simulink model "operational_space_inverse_dynamics"  (R2024b)
settings: Solver=VariableStepAuto  StartTime=0.0  StopTime=24*5+6  RelTol=1e-3
undefined symbols (not defined in the file): Kd_op, Ki_op, Kp_op, ml, q0, Tc
libraries: slpidlib x1
settings Model: Creator=storm  LastModifiedBy=giaco
settings OptimizationCC: ReuseModelBlockBuffer=off
settings DebuggingCC: UnconnectedInputMsg=warning  UnconnectedOutputMsg=warning  UnconnectedLineMsg=warning
settings ModelReferenceCC: EnableRefExpFcnMdlSchedulingChecks=on
settings RTWCC: GPUComputeCapability=3.5  DLArmComputeVersion=19.05

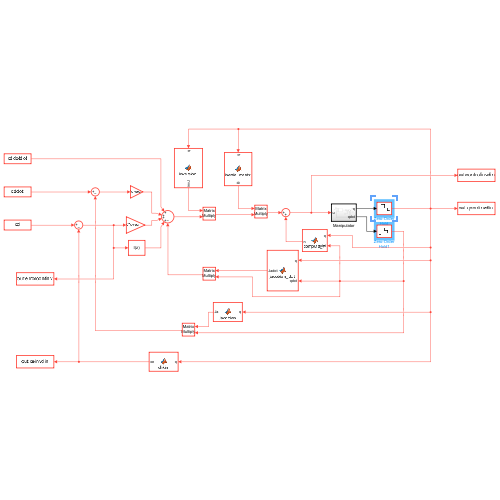
[thumbnail: Simulink's stored preview of the top-level diagram]
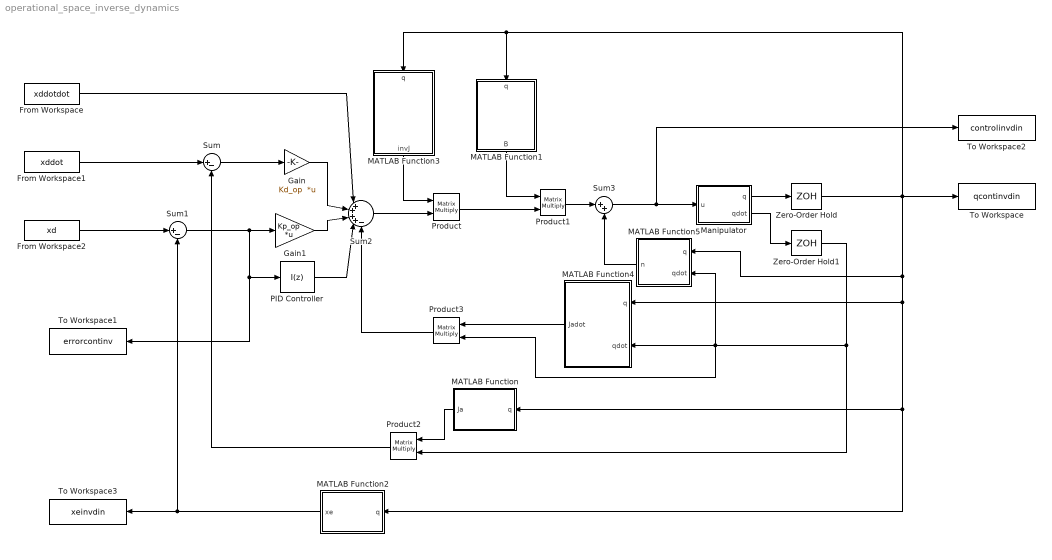
== system operational_space_inverse_dynamics ==
  From Workspace : FromWorkspace  VariableName=xddotdot  SampleTime=Tc
  From Workspace1 : FromWorkspace  VariableName=xddot  SampleTime=Tc
  From Workspace2 : FromWorkspace  VariableName=xd  SampleTime=Tc
  Gain : Gain  Gain=Kd_op  Multiplication=Matrix(K*u) (u vector)
  Gain1 : Gain  Gain=Kp_op  Multiplication=Matrix(K*u) (u vector)
  MATLAB Function : MATLAB Function  TreatAsAtomicUnit=on
  MATLAB Function1 : MATLAB Function  TreatAsAtomicUnit=on
  MATLAB Function2 : MATLAB Function  TreatAsAtomicUnit=on
  MATLAB Function3 : MATLAB Function  TreatAsAtomicUnit=on
  MATLAB Function4 : MATLAB Function  TreatAsAtomicUnit=on
  MATLAB Function5 : MATLAB Function  TreatAsAtomicUnit=on
  Manipulator : Subsystem
  PID Controller : slpidlib/PID Controller  Controller=I  Form=Parallel  TimeDomain=Discrete-time  UseExternalTs=off  SampleTime=-1  IntegratorMethod=Forward Euler  FilterMethod=Forward Euler  ControllerParametersSource=internal  P=1  I=diag(Ki_op)  UseKiTs=off  D=0  UseExternalDerivativeSource=off  N=100  UseFilter=on  TunerSelectOption=Transfer Function Based (PID Tuner App)  InitialConditionSource=internal  InitialConditionForIntegrator=0  InitialConditionForFilter=0  DifferentiatorICPrevScaledInput=0  ExternalReset=none  TrackingMode=off  Kt=1  LimitOutput=off  SatLimitsSource=internal  UpperSaturationLimit=inf  LowerSaturationLimit=-inf  LinearizeAsGain=on  AntiWindupMode=none  Kb=1  LimitIntegrator=off  UpperIntegratorSaturationLimit=inf  LowerIntegratorSaturationLimit=-inf  POutMin=[]  POutMax=[]  IOutMin=[]  IOutMax=[]  DOutMin=[]  DOutMax=[]  NOutMin=[]  NOutMax=[]  SumOutMin=[]  SumOutMax=[]  SaturationOutMin=[]  SaturationOutMax=[]  PParamMin=[]  PParamMax=[]  IParamMin=[]  IParamMax=[]  DParamMin=[]  DParamMax=[]  NParamMin=[]  NParamMax=[]  KbParamMin=[]  KbParamMax=[]  KtParamMin=[]  KtParamMax=[]  KbOutMin=[]  KbOutMax=[]  KtOutMin=[]  KtOutMax=[]  IntegratorOutMin=[]  IntegratorOutMax=[]  FilterOutMin=[]  FilterOutMax=[]  SumI1OutMin=[]  SumI1OutMax=[]  SumI2OutMin=[]  SumI2OutMax=[]  SumI3OutMin=[]  SumI3OutMax=[]  SumI4OutMin=[]  SumI4OutMax=[]  SumDOutMin=[]  SumDOutMax=[]  DifferentiatorOutMin=[]  DifferentiatorOutMax=[]  FilterDiffOutCoefMin=[]  FilterDiffOutCoefMax=[]  ReciprocalOutMin=[]  ReciprocalOutMax=[]  SumDenOutMin=[]  SumDenOutMax=[]  SumNumOutMin=[]  SumNumOutMax=[]  DivideOutMin=[]  DivideOutMax=[]  UdiffTsProdOutMin=[]  UdiffTsProdOutMax=[]  NTsProdOutMin=[]  NTsProdOutMax=[]  UintegralTsProdOutMin=[]  UintegralTsProdOutMax=[]  UngainTsProdOutMin=[]  UngainTsProdOutMax=[]  ClampingZeroOutDataTypeStr=Inherit: Inherit via back propagation  ClampingZeroOutMin=[]  ClampingZeroOutMax=[]  FilterDenConstantOutDataTypeStr=Inherit: Inherit via back propagation  FilterDenConstantOutMin=[]  FilterDenConstantOutMax=[]  PCopyOutDataTypeStr=Inherit: Inherit via back propagation  PCopyOutMin=[]  PCopyOutMax=[]  NCopyOutDataTypeStr=Inherit: Inherit via back propagation  NCopyOutMin=[]  NCopyOutMax=[]  IntegratorContinuousStateAttributes=''  IntegratorStateMustResolveToSignalObject=off  IntegratorRTWStateStorageClass=Auto  FilterContinuousStateAttributes=''  FilterStateMustResolveToSignalObject=off  FilterRTWStateStorageClass=Auto  ParallelPVariant=Disabled  IdealPVariant=Disabled  IVariant=InternalParameters  DVariant=Disabled  IntegratorVariant=Discrete  SatVariant=Disabled  AWVariant=Passthrough  PCopyVariant=Disabled  TRVariant=Disabled  FdbkBlocksVariant=Forward  IdealPFdbkVariant=Disabled  SatFdbkVariant=Disabled  DerivativeFilterVariant=Disabled  NVariant=Disabled  NCopyVariant=Disabled_SignalSpec  FilterICVariant=Disabled  IntegratorICVariant=InternalICs  ExternalResetVariant=Disabled  TRSumVariant=Passthrough  SumFdbkVariant=Disabled  SumVariant=Passthrough_I  TsampFilterVariant=InternalTs  TsampNgainVariant=Passthrough  TsampIntegralVariant=Disabled_SignalSpec  ExternalSaturationOutDataTypeStr=Inherit: Same as second input  DerivativeSourceVariant=Disabled  PreIntVariant=InternalPreInt
  Product{,1..3} (4 alike) : Product  Multiplication=Matrix(*)
  Sum : Sum  Inputs=|+-
  Sum1 : Sum  Inputs=|+-
  Sum2 : Sum  Inputs=|++++-
  Sum3 : Sum  Inputs=|++
  To Workspace : ToWorkspace  VariableName=qcontinvdin  SaveFormat=Structure With Time  SampleTime=-1
  To Workspace1 : ToWorkspace  VariableName=errorcontinv  SaveFormat=Structure With Time  SampleTime=-1
  To Workspace2 : ToWorkspace  VariableName=controlinvdin  SaveFormat=Structure With Time  SampleTime=-1
  To Workspace3 : ToWorkspace  VariableName=xeinvdin  SaveFormat=Structure With Time  SampleTime=-1
  Zero-Order Hold : ZeroOrderHold  SampleTime=Tc
  Zero-Order Hold1 : ZeroOrderHold  SampleTime=Tc
  wires:
  From Workspace1/1 -> Sum/1
  From Workspace2/1 -> Sum1/1
  Sum1/1 -> PID Controller/1, To Workspace1/1, Gain1/1
  Sum/1 -> Gain/1
  From Workspace/1 -> Sum2/1
  MATLAB Function3/1(invJ) -> Product/1
  Sum2/1 -> Product/2
  MATLAB Function1/1(B) -> Product1/1
  Product/1 -> Product1/2
  Product1/1 -> Sum3/1
  Manipulator/1(q) -> Zero-Order Hold/1
  Zero-Order Hold/1 -> MATLAB Function3/1(q), MATLAB Function1/1(q), MATLAB Function5/1(q), MATLAB Function4/1(q), MATLAB Function/1(q), MATLAB Function2/1(q), To Workspace/1
  MATLAB Function/1(Ja) -> Product2/1
  Product2/1 -> Sum/2
  MATLAB Function2/1(xe) -> Sum1/2, To Workspace3/1
  MATLAB Function4/1(Jadot) -> Product3/1
  Product3/1 -> Sum2/5
  MATLAB Function5/1(n) -> Sum3/2
  Gain/1 -> Sum2/2
  Gain1/1 -> Sum2/3
  Sum3/1 -> To Workspace2/1, Manipulator/1(u)
  Manipulator/2(qdot) -> Zero-Order Hold1/1
  Zero-Order Hold1/1 -> Product3/2, MATLAB Function5/2(qdot), MATLAB Function4/2(qdot), Product2/2
  PID Controller/1 -> Sum2/4

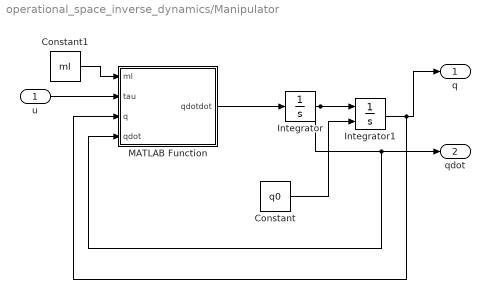
== system operational_space_inverse_dynamics/Manipulator ==
  u : Inport
  Constant : Constant  Value=q0
  Constant1 : Constant  Value=ml
  Integrator : Integrator  InitialCondition=[0 0 0 0]'
  Integrator1 : Integrator  InitialConditionSource=external
  MATLAB Function : MATLAB Function  TreatAsAtomicUnit=on
  q : Outport
  qdot : Outport  Port=2
  wires:
  u/1 -> MATLAB Function/2(tau)
  Integrator/1 -> MATLAB Function/4(qdot), qdot/1, Integrator1/1
  Constant/1 -> Integrator1/2
  Integrator1/1 -> MATLAB Function/3(q), q/1
  Constant1/1 -> MATLAB Function/1(ml)
  MATLAB Function/1(qdotdot) -> Integrator/1

== matlab function operational_space_inverse_dynamics/MATLAB Function2 ==
  data: q input; xe output
function xe = dirkin(q)
% Pose in base coordinates, ordered as [x; y; z; phi].
a1=0.5;
a2=a1;
d0=1;

xe=[a1*cos(q(1))+a2*cos(q(1)+q(2));...
    a1*sin(q(1))+a2*sin(q(1)+q(2));...
    d0+q(3);...
    q(1)+q(2)+q(4)];
end

== matlab function operational_space_inverse_dynamics/MATLAB Function ==
  data: q input; Ja output
function Ja = Jacobian(q)
% Map joint rates to [x_dot; y_dot; z_dot; phi_dot].
a1=0.5;
a2=a1;
d0=1;

Ja= [-a1*sin(q(1))-a2*sin(q(1)+q(2)),-a2*sin(q(1)+q(2)),0,0;...
    a1*cos(q(1))+a2*cos(q(1)+q(2)),a2*cos(q(1)+q(2)),0,0;...
    0,0,1,0;...
    1,1,0,1];
end

== matlab function operational_space_inverse_dynamics/MATLAB Function4 ==
  data: q input; Jadot output; qdot input
function Jadot = jacobian_dot(q,qdot)
% Only the planar rows change with the joint angles.

a1=0.5;
a2=a1;

Jadot= [qdot(1)*(-a1*cos(q(1)))-(qdot(1)+qdot(2))*a2*cos(q(1)+q(2)),(qdot(1)+qdot(2))*(-a2*cos(q(1)+q(2))),0,0;...
    qdot(1)*(-a1*sin(q(1)))-(qdot(1)+qdot(2))*a2*sin(q(1)+q(2)),(qdot(1)+qdot(2))*(-a2*sin(q(1)+q(2))),0,0;...
    0,0,0,0;...
    0,0,0,0];

end

== matlab function operational_space_inverse_dynamics/MATLAB Function3 ==
  data: invJ output; q input
function invJ=inversion(q)
% Map the full pose correction back to joint space.

a1=0.5;
a2=a1;

J = [-a1*sin(q(1))-a2*sin(q(1)+q(2)),-a2*sin(q(1)+q(2)),0,0;...
      a1*cos(q(1))+a2*cos(q(1)+q(2)),a2*cos(q(1)+q(2)),0,0;...
      0,0,1,0;...
      1,1,0,1];

invJ=J^-1;

end

== matlab function operational_space_inverse_dynamics/MATLAB Function1 ==
  data: q input; B output
function B = inertia_matrix(q)
% Joint-space inertia for the controller model.

a1=0.5;
a2=0.5;
l1=0.25;
l2=0.25;
ml1=20;
ml2=20;
ml3=10;
Il1=4;
Il2=4;
Il4=1;
kr1=1;
kr2=1;
kr3=50;
kr4=20;
Im1=0.01;
Im2=0.01;
Im3=0.005;
Im4=0.001;

mhe=0; % Payload mass parameter [kg]

% Link and rotor Jacobians used to assemble the inertia matrix.
Jpl1=[-l1*sin(q(1)) 0 0 0;
    l1*cos(q(1)) 0 0 0;
    0 0 0 0];

Jpl2=[-a1*sin(q(1))-l2*sin(q(1)+q(2)),-l2*sin(q(1)+q(2)),0,0;
    a1*cos(q(1))+l2*cos(q(1)+q(2)),l2*cos(q(1)+q(2)),0,0;
    0,0,0,0];

Jpl4=[-a1*sin(q(1))-a2*sin(q(1)+q(2)),-a2*sin(q(1)+q(2)),0,0;
    a1*cos(q(1))+a2*cos(q(1)+q(2)),a2*cos(q(1)+q(2)),0,0;
    0,0,1,0];

Jol1=[zeros(2,4);
    1 0 0 0];

Jol2=[zeros(2,4);
    1 1 0 0];

Jol4=[zeros(2,4);
    1 1 0 1];

Jom1=[zeros(2,4);
    kr1 0 0 0];

Jom2=[zeros(2,4);
    1 kr2 0 0];

Jom3=[zeros(2,4);
    1 1 kr3 0];

Jom4=[zeros(2,4);
    1 1 0 kr4];

B=ml1*(Jpl1'*Jpl1)+Jol1'*Il1*Jol1+Jom1'*Im1*Jom1...
    +ml2*(Jpl2'*Jpl2)+Jol2'*Il2*Jol2+Jom2'*Im2*Jom2...
    +Jom3'*Im3*Jom3...
    +(mhe+ml3)*(Jpl4'*Jpl4)+Jol4'*Il4*Jol4+Jom4'*Im4*Jom4;

end

== matlab function operational_space_inverse_dynamics/MATLAB Function5 ==
  data: q input; n output; qdot input
function n = compute_n(q,qdot)
% Add the velocity and gravity terms used in inverse dynamics.

a1=0.5;
a2=0.5;
l1=0.25;
l2=0.25;
ml1=20;
ml2=20;
ml3=10;
Il1=4;
Il2=4;
Il4=1;
kr1=1;
kr2=1;
kr3=50;
kr4=20;
Im1=0.01;
Im2=0.01;
Im3=0.005;
Im4=0.001;
Fm1=0.00005;
Fm2=0.00005;
Fm3=0.01;
Fm4=0.005;

mhe=0; % Payload mass parameter [kg]

% Link and rotor Jacobians used to assemble the inertia matrix.
Jpl1=[-l1*sin(q(1)) 0 0 0;
       l1*cos(q(1)) 0 0 0;
       0 0 0 0];

Jpl2=[-a1*sin(q(1))-l2*sin(q(1)+q(2)),-l2*sin(q(1)+q(2)),0,0;
       a1*cos(q(1))+l2*cos(q(1)+q(2)),l2*cos(q(1)+q(2)),0,0;
       0,0,0,0];

Jpl4=[-a1*sin(q(1))-a2*sin(q(1)+q(2)),-a2*sin(q(1)+q(2)),0,0;
       a1*cos(q(1))+a2*cos(q(1)+q(2)),a2*cos(q(1)+q(2)),0,0;
       0,0,1,0];

Jol1=[zeros(2,4);
      1 0 0 0];

Jol2=[zeros(2,4);
      1 1 0 0];

Jol4=[zeros(2,4);
      1 1 0 1];

Jom1=[zeros(2,4);
      kr1 0 0 0];

Jom2=[zeros(2,4);
      1 kr2 0 0];

Jom3=[zeros(2,4);
      1 1 kr3 0];

Jom4=[zeros(2,4);
      1 1 0 kr4];

B=ml1*(Jpl1'*Jpl1)+Jol1'*Il1*Jol1+Jom1'*Im1*Jom1...
    +ml2*(Jpl2'*Jpl2)+Jol2'*Il2*Jol2+Jom2'*Im2*Jom2...
    +Jom3'*Im3*Jom3...
    +ml3*(Jpl4'*Jpl4)+Jol4'*Il4*Jol4+Jom4'*Im4*Jom4;

% Build the Coriolis matrix from the inertia derivatives.
c=zeros(4,4,4);

Jpl1dq1=[-l1*cos(q(1)) 0 0 0;
         -l1*sin(q(1)) 0 0 0;
          0 0 0 0];

Jpl1dq2=zeros(3,4);

Jpl2dq1=[-a1*cos(q(1))-l2*cos(q(1)+q(2)),-l2*cos(q(1)+q(2)),0,0;
         -a1*sin(q(1))-l2*sin(q(1)+q(2)),-l2*sin(q(1)+q(2)),0,0;
          0,0,0,0];

Jpl2dq2=[-l2*cos(q(1)+q(2)),-l2*cos(q(1)+q(2)),0,0;
         -l2*sin(q(1)+q(2)),-l2*sin(q(1)+q(2)),0,0;
          0,0,0,0];

Jpl4dq1=[-a1*cos(q(1))-a2*cos(q(1)+q(2)),-a2*cos(q(1)+q(2)),0,0;
         -a1*sin(q(1))-a2*sin(q(1)+q(2)),-a2*sin(q(1)+q(2)),0,0;
          0,0,0,0];

Jpl4dq2=[-a2*cos(q(1)+q(2)),-a2*cos(q(1)+q(2)),0,0;
         -a2*sin(q(1)+q(2)),-a2*sin(q(1)+q(2)),0,0;
          0,0,0,0];

dBdq1=ml1*(Jpl1dq1'*Jpl1+Jpl1'*Jpl1dq1)+ml2*(Jpl2dq1'*Jpl2+Jpl2'*Jpl2dq1)+ml3*(Jpl4dq1'*Jpl4+Jpl4'*Jpl4dq1);
dBdq2=ml1*(Jpl1dq2'*Jpl1+Jpl1'*Jpl1dq2)+ml2*(Jpl2dq2'*Jpl2+Jpl2'*Jpl2dq2)+ml3*(Jpl4dq2'*Jpl4+Jpl4'*Jpl4dq2);

c(1,1,2)=-ml2*a1*l2*sin(q(2))-ml3*a1*a2*sin(q(2));
c(1,2,2)=c(1,1,2);
c(2,1,1)=-c(1,1,2);

C=zeros(4,4);
    for i=1:4
        for j=1:4
            for k=1:4
                C(i,j)=c(i,j,k)*qdot(k);
            end
        end
    end

g = [0 0 9.81*(mhe+ml3) 0]';

Fv = diag([kr1^2*Fm1,kr2^2*Fm2,kr3^2*Fm3,kr4^2*Fm4]);

n = C*qdot+Fv*qdot+g;

== matlab function operational_space_inverse_dynamics/Manipulator/MATLAB Function ==
  data: ml input; qdotdot output; tau input; q input; qdot input
function qdotdot= Dinamica_diretta(ml,tau,q,qdot)
% Plant dynamics: subtract Coriolis, friction, and gravity before solving for acceleration.
a1=0.5;
a2=0.5;
l1=0.25;
l2=0.25;
ml1=20;
ml2=20;
ml3=10;
Il1=4;
Il2=4;
Il4=1;
kr1=1;
kr2=1;
kr3=50;
kr4=20;
Im1=0.01;
Im2=0.01;
Im3=0.005;
Im4=0.001;

Fm1=0.00005;
Fm2=0.00005;
Fm3=0.01;
Fm4=0.005;

mhe=4; % Payload mass parameter [kg]
% Link and rotor Jacobians used to assemble the inertia matrix.
Jpl1=[-l1*sin(q(1)) 0 0 0;
    l1*cos(q(1)) 0 0 0;
    0 0 0 0];

Jpl2=[-a1*sin(q(1))-l2*sin(q(1)+q(2)),-l2*sin(q(1)+q(2)),0,0;
    a1*cos(q(1))+l2*cos(q(1)+q(2)),l2*cos(q(1)+q(2)),0,0;
    0,0,0,0];

Jpl4=[-a1*sin(q(1))-a2*sin(q(1)+q(2)),-a2*sin(q(1)+q(2)),0,0;
    a1*cos(q(1))+a2*cos(q(1)+q(2)),a2*cos(q(1)+q(2)),0,0;
    0,0,1,0];

Jol1=[zeros(2,4);
    1 0 0 0];

Jol2=[zeros(2,4);
    1 1 0 0];

Jol4=[zeros(2,4);
    1 1 0 1];

Jom1=[zeros(2,4);
    kr1 0 0 0];

Jom2=[zeros(2,4);
    1 kr2 0 0];

Jom3=[zeros(2,4);
    1 1 kr3 0];

Jom4=[zeros(2,4);
    1 1 0 kr4];

B=ml1*(Jpl1'*Jpl1)+Jol1'*Il1*Jol1+Jom1'*Im1*Jom1...
    +ml2*(Jpl2'*Jpl2)+Jol2'*Il2*Jol2+Jom2'*Im2*Jom2...
    +Jom3'*Im3*Jom3...
    +(ml+ml3)*(Jpl4'*Jpl4)+Jol4'*Il4*Jol4+Jom4'*Im4*Jom4;

c=zeros(4,4,4);

Jpl1dq1=[-l1*cos(q(1)) 0 0 0;
    -l1*sin(q(1)) 0 0 0;
    0 0 0 0];

Jpl1dq2=zeros(3,4);

Jpl2dq1=[-a1*cos(q(1))-l2*cos(q(1)+q(2)),-l2*cos(q(1)+q(2)),0,0;
    -a1*sin(q(1))-l2*sin(q(1)+q(2)),-l2*sin(q(1)+q(2)),0,0;
    0,0,0,0];

Jpl2dq2=[-l2*cos(q(1)+q(2)),-l2*cos(q(1)+q(2)),0,0;
    -l2*sin(q(1)+q(2)),-l2*sin(q(1)+q(2)),0,0;
    0,0,0,0];

Jpl4dq1=[-a1*cos(q(1))-a2*cos(q(1)+q(2)),-a2*cos(q(1)+q(2)),0,0;
    -a1*sin(q(1))-a2*sin(q(1)+q(2)),-a2*sin(q(1)+q(2)),0,0;
    0,0,0,0];

Jpl4dq2=[-a2*cos(q(1)+q(2)),-a2*cos(q(1)+q(2)),0,0;
    -a2*sin(q(1)+q(2)),-a2*sin(q(1)+q(2)),0,0;
    0,0,0,0];

dBdq1=ml1*(Jpl1dq1'*Jpl1+Jpl1'*Jpl1dq1)+ml2*(Jpl2dq1'*Jpl2+Jpl2'*Jpl2dq1)+ml3*(Jpl4dq1'*Jpl4+Jpl4'*Jpl4dq1);
dBdq2=ml1*(Jpl1dq2'*Jpl1+Jpl1'*Jpl1dq2)+ml2*(Jpl2dq2'*Jpl2+Jpl2'*Jpl2dq2)+ml3*(Jpl4dq2'*Jpl4+Jpl4'*Jpl4dq2);

c(1,1,2)=-ml2*a1*l2*sin(q(2))-ml3*a1*a2*sin(q(2));
c(1,2,2)=c(1,1,2);
c(2,1,1)=-c(1,1,2);

C=zeros(4,4);
    for i=1:4
        for j=1:4
            for k=1:4
                C(i,j)=c(i,j,k)*qdot(k);
            end
        end
    end

g=[0 0 9.81*(ml+ml3) 0]';

Fv=diag([kr1^2*Fm1,kr2^2*Fm2,kr3^2*Fm3,kr4^2*Fm4]);
qdotdot=inv(B)*(tau-C*qdot-Fv*qdot-g);
end
